simulink model "Hexapod_dev"  (R2026a)
settings: Solver=daessc  StopTime=ref.t(end)  FixedStep=2e-5
InitFcn:
  | startup
model workspace: external: MATLAB File Hexapod_DataFile.m (data not in the file)
undefined symbols (not defined in the file): ref, robot, smiData, X, Y, Z
libraries: sm_lib x805, nesl_utility x43
(part 14 of 15)

== system Hexapod_dev/Spherical Joints/HeimJoint_No_Ball_1_RIGID4/x6960T432_Super_Swivel_Ball_Joint_Rod_End_No_Ball_1_RIGID ==
  ReferenceFrame : sm_lib/Frames and Transforms/Reference Frame
  Solid : sm_lib/Body Elements/File Solid  ExtGeomFileName=6960T432_Super-Swivel Ball Joint Rod End No Ball_6960T432_sldprt.STEP  UnitType=FromFile  ExtGeomFileUnits=m  StepReaderType=HEX  ExportConvexHullGeometry=off  InertiaType=Custom  BasedOnType=DensityFromFile  Density=1000  DensityUnits=kg/m^3  Mass=smiData.Solid(21).mass  MassUnits=kg  CenterOfMass=smiData.Solid(21).CoM  CenterOfMassUnits=in  MomentsOfInertia=smiData.Solid(21).MoI  MomentsOfInertiaUnits=kg*in^2  ProductsOfInertia=smiData.Solid(21).PoI  ProductsOfInertiaUnits=kg*in^2  GraphicType=FromGeometry  MarkerShape=Sphere  MarkerSize=10  GraphicVisPropType=SimpleVisualProperties  GraphicDiffuseColor=smiData.Solid(21).color  GraphicOpacity=smiData.Solid(21).opacity  GraphicSpecularColor=[0.5 0.5 0.5 1.0]  GraphicAmbientColor=[0.15 0.15 0.15 1.0]  GraphicEmissiveColor=[0.0 0.0 0.0 1.0]  GraphicShininess=75  DoExposeReferenceFrame=on  SerializedFrames=|
      | <Frames>
      | 
      |   <Frame>
      |     <Id>Frame1</Id>
      |     <Value>
      |       <Name>T</Name>
      |       <Origin>
      |         <Source>GeometricFeature</Source>
      |         <FeatureName>spherical surface 2</FeatureName>
      |       </Origin>
      |       <PrimaryAxis>
      |         <DefinedDirection>+Z</DefinedDirection>
      |         <Source>ReferenceFrame</Source>
      |         <SourceDirection>+Z</SourceDirection>
      |         <FeatureName></FeatureName>
      |       </PrimaryAxis>
      |       <SecondaryAxis>
      |         <DefinedDirection>+X</DefinedDirection>
      |         <Source>GeometricFeature</Source>
      |         <SourceDirection>+X</SourceDirection>
      |         <FeatureName>segment 75</FeatureName>
      |       </SecondaryAxis>
      |     </Value>
      |   </Frame>
      | 
      | </Frames>
  F : PMIOPort  Side=Left
  T : PMIOPort  Port=2  Side=Left
  connections:
  ReferenceFrame/RConn1 -- Solid/RConn1 -- F/RConn1
  T/RConn1 -- Solid/LConn1

== system Hexapod_dev/Spherical Joints/HeimJoint_No_Ball_1_RIGID4/x8422N111_18_8_Stainless_Steel_Turnbuckle_Style_Connecting_Rod_1_RIGID ==
  ReferenceFrame : sm_lib/Frames and Transforms/Reference Frame
  Solid : sm_lib/Body Elements/File Solid  ExtGeomFileName=8422N111_18-8 Stainless Steel Turnbuckle-Style Connecting Rod_8422N111_sldprt.STEP  UnitType=FromFile  ExtGeomFileUnits=m  StepReaderType=HEX  ExportConvexHullGeometry=off  InertiaType=Custom  BasedOnType=DensityFromFile  Density=1000  DensityUnits=kg/m^3  Mass=smiData.Solid(19).mass  MassUnits=kg  CenterOfMass=smiData.Solid(19).CoM  CenterOfMassUnits=in  MomentsOfInertia=smiData.Solid(19).MoI  MomentsOfInertiaUnits=kg*in^2  ProductsOfInertia=smiData.Solid(19).PoI  ProductsOfInertiaUnits=kg*in^2  GraphicType=FromGeometry  MarkerShape=Sphere  MarkerSize=10  GraphicVisPropType=SimpleVisualProperties  GraphicDiffuseColor=smiData.Solid(19).color  GraphicOpacity=smiData.Solid(19).opacity  GraphicSpecularColor=[0.5 0.5 0.5 1.0]  GraphicAmbientColor=[0.15 0.15 0.15 1.0]  GraphicEmissiveColor=[0.0 0.0 0.0 1.0]  GraphicShininess=75  DoExposeReferenceFrame=on  SerializedFrames=<Frames/>
  F : PMIOPort  Side=Left
  connections:
  Solid/RConn1 -- ReferenceFrame/RConn1 -- F/RConn1

== system Hexapod_dev/Spherical Joints/HeimJoint_No_Ball_1_RIGID5/x6960T431_Super_Swivel_Ball_Joint_Rod_End_No_Ball_1_RIGID ==
  ReferenceFrame : sm_lib/Frames and Transforms/Reference Frame
  Solid : sm_lib/Body Elements/File Solid  ExtGeomFileName=6960T431_Super-Swivel Ball Joint Rod End No Ball_6960T431_sldprt.STEP  UnitType=FromFile  ExtGeomFileUnits=m  StepReaderType=HEX  ExportConvexHullGeometry=off  InertiaType=Custom  BasedOnType=DensityFromFile  Density=1000  DensityUnits=kg/m^3  Mass=smiData.Solid(20).mass  MassUnits=kg  CenterOfMass=smiData.Solid(20).CoM  CenterOfMassUnits=in  MomentsOfInertia=smiData.Solid(20).MoI  MomentsOfInertiaUnits=kg*in^2  ProductsOfInertia=smiData.Solid(20).PoI  ProductsOfInertiaUnits=kg*in^2  GraphicType=FromGeometry  MarkerShape=Sphere  MarkerSize=10  GraphicVisPropType=SimpleVisualProperties  GraphicDiffuseColor=smiData.Solid(20).color  GraphicOpacity=smiData.Solid(20).opacity  GraphicSpecularColor=[0.5 0.5 0.5 1.0]  GraphicAmbientColor=[0.15 0.15 0.15 1.0]  GraphicEmissiveColor=[0.0 0.0 0.0 1.0]  GraphicShininess=75  DoExposeReferenceFrame=on  SerializedFrames=|
      | <Frames>
      | 
      |   <Frame>
      |     <Id>Frame1</Id>
      |     <Value>
      |       <Name>B</Name>
      |       <Origin>
      |         <Source>GeometricFeature</Source>
      |         <FeatureName>circular curve 99</FeatureName>
      |       </Origin>
      |       <PrimaryAxis>
      |         <DefinedDirection>+Z</DefinedDirection>
      |         <Source>ReferenceFrame</Source>
      |         <SourceDirection>+Z</SourceDirection>
      |         <FeatureName></FeatureName>
      |       </PrimaryAxis>
      |       <SecondaryAxis>
      |         <DefinedDirection>-X</DefinedDirection>
      |         <Source>GeometricFeature</Source>
      |         <SourceDirection>+X</SourceDirection>
      |         <FeatureName>segment 73</FeatureName>
      |       </SecondaryAxis>
      |     </Value>
      |   </Frame>
      | 
      | </Frames>
  F : PMIOPort  Side=Left
  BO : PMIOPort  Port=2  Side=Left
  connections:
  ReferenceFrame/RConn1 -- Solid/RConn1 -- F/RConn1
  BO/RConn1 -- Solid/LConn1

== system Hexapod_dev/Spherical Joints/HeimJoint_No_Ball_1_RIGID5/x6960T432_Super_Swivel_Ball_Joint_Rod_End_No_Ball_1_RIGID ==
  ReferenceFrame : sm_lib/Frames and Transforms/Reference Frame
  Solid : sm_lib/Body Elements/File Solid  ExtGeomFileName=6960T432_Super-Swivel Ball Joint Rod End No Ball_6960T432_sldprt.STEP  UnitType=FromFile  ExtGeomFileUnits=m  StepReaderType=HEX  ExportConvexHullGeometry=off  InertiaType=Custom  BasedOnType=DensityFromFile  Density=1000  DensityUnits=kg/m^3  Mass=smiData.Solid(21).mass  MassUnits=kg  CenterOfMass=smiData.Solid(21).CoM  CenterOfMassUnits=in  MomentsOfInertia=smiData.Solid(21).MoI  MomentsOfInertiaUnits=kg*in^2  ProductsOfInertia=smiData.Solid(21).PoI  ProductsOfInertiaUnits=kg*in^2  GraphicType=FromGeometry  MarkerShape=Sphere  MarkerSize=10  GraphicVisPropType=SimpleVisualProperties  GraphicDiffuseColor=smiData.Solid(21).color  GraphicOpacity=smiData.Solid(21).opacity  GraphicSpecularColor=[0.5 0.5 0.5 1.0]  GraphicAmbientColor=[0.15 0.15 0.15 1.0]  GraphicEmissiveColor=[0.0 0.0 0.0 1.0]  GraphicShininess=75  DoExposeReferenceFrame=on  SerializedFrames=|
      | <Frames>
      | 
      |   <Frame>
      |     <Id>Frame1</Id>
      |     <Value>
      |       <Name>T</Name>
      |       <Origin>
      |         <Source>GeometricFeature</Source>
      |         <FeatureName>spherical surface 2</FeatureName>
      |       </Origin>
      |       <PrimaryAxis>
      |         <DefinedDirection>+Z</DefinedDirection>
      |         <Source>ReferenceFrame</Source>
      |         <SourceDirection>+Z</SourceDirection>
      |         <FeatureName></FeatureName>
      |       </PrimaryAxis>
      |       <SecondaryAxis>
      |         <DefinedDirection>+X</DefinedDirection>
      |         <Source>GeometricFeature</Source>
      |         <SourceDirection>+X</SourceDirection>
      |         <FeatureName>segment 75</FeatureName>
      |       </SecondaryAxis>
      |     </Value>
      |   </Frame>
      | 
      | </Frames>
  F : PMIOPort  Side=Left
  T : PMIOPort  Port=2  Side=Left
  connections:
  ReferenceFrame/RConn1 -- Solid/RConn1 -- F/RConn1
  T/RConn1 -- Solid/LConn1

== system Hexapod_dev/Spherical Joints/HeimJoint_No_Ball_1_RIGID5/x8422N111_18_8_Stainless_Steel_Turnbuckle_Style_Connecting_Rod_1_RIGID ==
  ReferenceFrame : sm_lib/Frames and Transforms/Reference Frame
  Solid : sm_lib/Body Elements/File Solid  ExtGeomFileName=8422N111_18-8 Stainless Steel Turnbuckle-Style Connecting Rod_8422N111_sldprt.STEP  UnitType=FromFile  ExtGeomFileUnits=m  StepReaderType=HEX  ExportConvexHullGeometry=off  InertiaType=Custom  BasedOnType=DensityFromFile  Density=1000  DensityUnits=kg/m^3  Mass=smiData.Solid(19).mass  MassUnits=kg  CenterOfMass=smiData.Solid(19).CoM  CenterOfMassUnits=in  MomentsOfInertia=smiData.Solid(19).MoI  MomentsOfInertiaUnits=kg*in^2  ProductsOfInertia=smiData.Solid(19).PoI  ProductsOfInertiaUnits=kg*in^2  GraphicType=FromGeometry  MarkerShape=Sphere  MarkerSize=10  GraphicVisPropType=SimpleVisualProperties  GraphicDiffuseColor=smiData.Solid(19).color  GraphicOpacity=smiData.Solid(19).opacity  GraphicSpecularColor=[0.5 0.5 0.5 1.0]  GraphicAmbientColor=[0.15 0.15 0.15 1.0]  GraphicEmissiveColor=[0.0 0.0 0.0 1.0]  GraphicShininess=75  DoExposeReferenceFrame=on  SerializedFrames=<Frames/>
  F : PMIOPort  Side=Left
  connections:
  Solid/RConn1 -- ReferenceFrame/RConn1 -- F/RConn1

== system Hexapod_dev/Spherical Joints/HeimJoint_No_Ball_1_RIGID6/x6960T431_Super_Swivel_Ball_Joint_Rod_End_No_Ball_1_RIGID ==
  ReferenceFrame : sm_lib/Frames and Transforms/Reference Frame
  Solid : sm_lib/Body Elements/File Solid  ExtGeomFileName=6960T431_Super-Swivel Ball Joint Rod End No Ball_6960T431_sldprt.STEP  UnitType=FromFile  ExtGeomFileUnits=m  StepReaderType=HEX  ExportConvexHullGeometry=off  InertiaType=Custom  BasedOnType=DensityFromFile  Density=1000  DensityUnits=kg/m^3  Mass=smiData.Solid(20).mass  MassUnits=kg  CenterOfMass=smiData.Solid(20).CoM  CenterOfMassUnits=in  MomentsOfInertia=smiData.Solid(20).MoI  MomentsOfInertiaUnits=kg*in^2  ProductsOfInertia=smiData.Solid(20).PoI  ProductsOfInertiaUnits=kg*in^2  GraphicType=FromGeometry  MarkerShape=Sphere  MarkerSize=10  GraphicVisPropType=SimpleVisualProperties  GraphicDiffuseColor=smiData.Solid(20).color  GraphicOpacity=smiData.Solid(20).opacity  GraphicSpecularColor=[0.5 0.5 0.5 1.0]  GraphicAmbientColor=[0.15 0.15 0.15 1.0]  GraphicEmissiveColor=[0.0 0.0 0.0 1.0]  GraphicShininess=75  DoExposeReferenceFrame=on  SerializedFrames=|
      | <Frames>
      | 
      |   <Frame>
      |     <Id>Frame1</Id>
      |     <Value>
      |       <Name>B</Name>
      |       <Origin>
      |         <Source>GeometricFeature</Source>
      |         <FeatureName>circular curve 99</FeatureName>
      |       </Origin>
      |       <PrimaryAxis>
      |         <DefinedDirection>+Z</DefinedDirection>
      |         <Source>ReferenceFrame</Source>
      |         <SourceDirection>+Z</SourceDirection>
      |         <FeatureName></FeatureName>
      |       </PrimaryAxis>
      |       <SecondaryAxis>
      |         <DefinedDirection>-X</DefinedDirection>
      |         <Source>GeometricFeature</Source>
      |         <SourceDirection>+X</SourceDirection>
      |         <FeatureName>segment 73</FeatureName>
      |       </SecondaryAxis>
      |     </Value>
      |   </Frame>
      | 
      | </Frames>
  F : PMIOPort  Side=Left
  B : PMIOPort  Port=2  Side=Right
  connections:
  ReferenceFrame/RConn1 -- Solid/RConn1 -- F/RConn1
  B/RConn1 -- Solid/LConn1

== system Hexapod_dev/Spherical Joints/HeimJoint_No_Ball_1_RIGID6/x6960T432_Super_Swivel_Ball_Joint_Rod_End_No_Ball_1_RIGID ==
  ReferenceFrame : sm_lib/Frames and Transforms/Reference Frame
  Solid : sm_lib/Body Elements/File Solid  ExtGeomFileName=6960T432_Super-Swivel Ball Joint Rod End No Ball_6960T432_sldprt.STEP  UnitType=FromFile  ExtGeomFileUnits=m  StepReaderType=HEX  ExportConvexHullGeometry=off  InertiaType=Custom  BasedOnType=DensityFromFile  Density=1000  DensityUnits=kg/m^3  Mass=smiData.Solid(21).mass  MassUnits=kg  CenterOfMass=smiData.Solid(21).CoM  CenterOfMassUnits=in  MomentsOfInertia=smiData.Solid(21).MoI  MomentsOfInertiaUnits=kg*in^2  ProductsOfInertia=smiData.Solid(21).PoI  ProductsOfInertiaUnits=kg*in^2  GraphicType=FromGeometry  MarkerShape=Sphere  MarkerSize=10  GraphicVisPropType=SimpleVisualProperties  GraphicDiffuseColor=smiData.Solid(21).color  GraphicOpacity=smiData.Solid(21).opacity  GraphicSpecularColor=[0.5 0.5 0.5 1.0]  GraphicAmbientColor=[0.15 0.15 0.15 1.0]  GraphicEmissiveColor=[0.0 0.0 0.0 1.0]  GraphicShininess=75  DoExposeReferenceFrame=on  SerializedFrames=|
      | <Frames>
      | 
      |   <Frame>
      |     <Id>Frame1</Id>
      |     <Value>
      |       <Name>T</Name>
      |       <Origin>
      |         <Source>GeometricFeature</Source>
      |         <FeatureName>spherical surface 2</FeatureName>
      |       </Origin>
      |       <PrimaryAxis>
      |         <DefinedDirection>+Z</DefinedDirection>
      |         <Source>ReferenceFrame</Source>
      |         <SourceDirection>+Z</SourceDirection>
      |         <FeatureName></FeatureName>
      |       </PrimaryAxis>
      |       <SecondaryAxis>
      |         <DefinedDirection>+X</DefinedDirection>
      |         <Source>GeometricFeature</Source>
      |         <SourceDirection>+X</SourceDirection>
      |         <FeatureName>segment 75</FeatureName>
      |       </SecondaryAxis>
      |     </Value>
      |   </Frame>
      | 
      | </Frames>
  F : PMIOPort  Side=Left
  T : PMIOPort  Port=2  Side=Right
  connections:
  ReferenceFrame/RConn1 -- Solid/RConn1 -- F/RConn1
  T/RConn1 -- Solid/LConn1

== system Hexapod_dev/Spherical Joints/HeimJoint_No_Ball_1_RIGID6/x8422N111_18_8_Stainless_Steel_Turnbuckle_Style_Connecting_Rod_1_RIGID ==
  ReferenceFrame : sm_lib/Frames and Transforms/Reference Frame
  Solid : sm_lib/Body Elements/File Solid  ExtGeomFileName=8422N111_18-8 Stainless Steel Turnbuckle-Style Connecting Rod_8422N111_sldprt.STEP  UnitType=FromFile  ExtGeomFileUnits=m  StepReaderType=HEX  ExportConvexHullGeometry=off  InertiaType=Custom  BasedOnType=DensityFromFile  Density=1000  DensityUnits=kg/m^3  Mass=smiData.Solid(19).mass  MassUnits=kg  CenterOfMass=smiData.Solid(19).CoM  CenterOfMassUnits=in  MomentsOfInertia=smiData.Solid(19).MoI  MomentsOfInertiaUnits=kg*in^2  ProductsOfInertia=smiData.Solid(19).PoI  ProductsOfInertiaUnits=kg*in^2  GraphicType=FromGeometry  MarkerShape=Sphere  MarkerSize=10  GraphicVisPropType=SimpleVisualProperties  GraphicDiffuseColor=smiData.Solid(19).color  GraphicOpacity=smiData.Solid(19).opacity  GraphicSpecularColor=[0.5 0.5 0.5 1.0]  GraphicAmbientColor=[0.15 0.15 0.15 1.0]  GraphicEmissiveColor=[0.0 0.0 0.0 1.0]  GraphicShininess=75  DoExposeReferenceFrame=on  SerializedFrames=<Frames/>
  F : PMIOPort  Side=Left
  connections:
  Solid/RConn1 -- ReferenceFrame/RConn1 -- F/RConn1

== system Hexapod_dev/Spherical Joints/MotorRotor_a_1_RIGID/MotorRotor_1_RIGID ==
  Inertia : sm_lib/Body Elements/Inertia  InertiaType=Custom  Mass=0  MassUnits=kg  CenterOfMass=[0 0 0]  CenterOfMassUnits=m  MomentsOfInertia="[0 0  robot.motor.reflectedInertia]"  MomentsOfInertiaUnits=kg*m^2  ProductsOfInertia=[0 0 0]  ProductsOfInertiaUnits=kg*m^2  GraphicType=None  MarkerShape=Inertia  MarkerSize=20  GraphicVisPropType=SimpleVisualProperties  GraphicDiffuseColor=[0.5 0.5 0.5]  GraphicOpacity=1  GraphicSpecularColor=[0.5 0.5 0.5 1.0]  GraphicAmbientColor=[0.15 0.15 0.15 1.0]  GraphicEmissiveColor=[0.0 0.0 0.0 1.0]  GraphicShininess=75
  ReferenceFrame : sm_lib/Frames and Transforms/Reference Frame
  Solid : sm_lib/Body Elements/File Solid  ExtGeomFileName=MotorRotor_Default_sldprt.STEP  UnitType=FromFile  ExtGeomFileUnits=m  StepReaderType=HEX  ExportConvexHullGeometry=off  InertiaType=Custom  BasedOnType=DensityFromFile  Density=1000  DensityUnits=kg/m^3  Mass=smiData.Solid(16).mass  MassUnits=kg  CenterOfMass=smiData.Solid(16).CoM  CenterOfMassUnits=mm  MomentsOfInertia=smiData.Solid(16).MoI  MomentsOfInertiaUnits=kg*mm^2  ProductsOfInertia=smiData.Solid(16).PoI  ProductsOfInertiaUnits=kg*mm^2  GraphicType=FromGeometry  MarkerShape=Sphere  MarkerSize=10  GraphicVisPropType=SimpleVisualProperties  GraphicDiffuseColor=smiData.Solid(16).color  GraphicOpacity=smiData.Solid(16).opacity  GraphicSpecularColor=[0.5 0.5 0.5 1.0]  GraphicAmbientColor=[0.15 0.15 0.15 1.0]  GraphicEmissiveColor=[0.0 0.0 0.0 1.0]  GraphicShininess=75  DoExposeReferenceFrame=on  SerializedFrames=<Frames/>
  F : PMIOPort  Side=Left
  connections:
  ReferenceFrame/RConn1 -- F/RConn1 -- Inertia/RConn1 -- Solid/RConn1

== system Hexapod_dev/Spherical Joints/MotorRotor_a_1_RIGID/ServoArm_1_RIGID ==
  ReferenceFrame : sm_lib/Frames and Transforms/Reference Frame
  Solid : sm_lib/Body Elements/File Solid  ExtGeomFileName=ServoArm_Default_sldprt.STEP  UnitType=FromFile  ExtGeomFileUnits=m  StepReaderType=HEX  ExportConvexHullGeometry=off  InertiaType=Custom  BasedOnType=DensityFromFile  Density=1000  DensityUnits=kg/m^3  Mass=smiData.Solid(18).mass  MassUnits=kg  CenterOfMass=smiData.Solid(18).CoM  CenterOfMassUnits=in  MomentsOfInertia=smiData.Solid(18).MoI  MomentsOfInertiaUnits=kg*in^2  ProductsOfInertia=smiData.Solid(18).PoI  ProductsOfInertiaUnits=kg*in^2  GraphicType=FromGeometry  MarkerShape=Sphere  MarkerSize=10  GraphicVisPropType=SimpleVisualProperties  GraphicDiffuseColor=smiData.Solid(18).color  GraphicOpacity=smiData.Solid(18).opacity  GraphicSpecularColor=[0.5 0.5 0.5 1.0]  GraphicAmbientColor=[0.15 0.15 0.15 1.0]  GraphicEmissiveColor=[0.0 0.0 0.0 1.0]  GraphicShininess=75  DoExposeReferenceFrame=on  SerializedFrames=<Frames/>
  F : PMIOPort  Side=Left
  connections:
  Solid/RConn1 -- ReferenceFrame/RConn1 -- F/RConn1

== system Hexapod_dev/Spherical Joints/MotorRotor_a_1_RIGID/ball_1_RIGID ==
  ReferenceFrame : sm_lib/Frames and Transforms/Reference Frame
  Solid : sm_lib/Body Elements/File Solid  ExtGeomFileName=ball_6960T431_sldprt.STEP  UnitType=FromFile  ExtGeomFileUnits=m  StepReaderType=HEX  ExportConvexHullGeometry=off  InertiaType=Custom  BasedOnType=DensityFromFile  Density=1000  DensityUnits=kg/m^3  Mass=smiData.Solid(12).mass  MassUnits=kg  CenterOfMass=smiData.Solid(12).CoM  CenterOfMassUnits=in  MomentsOfInertia=smiData.Solid(12).MoI  MomentsOfInertiaUnits=kg*in^2  ProductsOfInertia=smiData.Solid(12).PoI  ProductsOfInertiaUnits=kg*in^2  GraphicType=FromGeometry  MarkerShape=Sphere  MarkerSize=10  GraphicVisPropType=SimpleVisualProperties  GraphicDiffuseColor=smiData.Solid(12).color  GraphicOpacity=smiData.Solid(12).opacity  GraphicSpecularColor=[0.5 0.5 0.5 1.0]  GraphicAmbientColor=[0.15 0.15 0.15 1.0]  GraphicEmissiveColor=[0.0 0.0 0.0 1.0]  GraphicShininess=75  DoExposeReferenceFrame=on  SerializedFrames=<Frames/>
  F : PMIOPort  Side=Left
  connections:
  Solid/RConn1 -- ReferenceFrame/RConn1 -- F/RConn1

== system Hexapod_dev/Spherical Joints/MotorRotor_a_1_RIGID/x90790A185_Black_Oxide_Steel_High_Heavy_Profile_Cap_Nut_1_RIGID ==
  ReferenceFrame : sm_lib/Frames and Transforms/Reference Frame
  Solid : sm_lib/Body Elements/File Solid  ExtGeomFileName=90790A185_Black-Oxide Steel High-Heavy-Profile Cap Nut_90790A185_sldprt.STEP  UnitType=FromFile  ExtGeomFileUnits=m  StepReaderType=HEX  ExportConvexHullGeometry=off  InertiaType=Custom  BasedOnType=DensityFromFile  Density=1000  DensityUnits=kg/m^3  Mass=smiData.Solid(13).mass  MassUnits=kg  CenterOfMass=smiData.Solid(13).CoM  CenterOfMassUnits=in  MomentsOfInertia=smiData.Solid(13).MoI  MomentsOfInertiaUnits=kg*in^2  ProductsOfInertia=smiData.Solid(13).PoI  ProductsOfInertiaUnits=kg*in^2  GraphicType=FromGeometry  MarkerShape=Sphere  MarkerSize=10  GraphicVisPropType=SimpleVisualProperties  GraphicDiffuseColor=smiData.Solid(13).color  GraphicOpacity=smiData.Solid(13).opacity  GraphicSpecularColor=[0.5 0.5 0.5 1.0]  GraphicAmbientColor=[0.15 0.15 0.15 1.0]  GraphicEmissiveColor=[0.0 0.0 0.0 1.0]  GraphicShininess=75  DoExposeReferenceFrame=on  SerializedFrames=<Frames/>
  F : PMIOPort  Side=Left
  connections:
  Solid/RConn1 -- ReferenceFrame/RConn1 -- F/RConn1

== system Hexapod_dev/Spherical Joints/MotorRotor_a_1_RIGID/x91259A628_Alloy_Steel_Shoulder_Screw_1_RIGID ==
  ReferenceFrame : sm_lib/Frames and Transforms/Reference Frame
  Solid : sm_lib/Body Elements/File Solid  ExtGeomFileName=91259A628_Alloy Steel Shoulder Screw_91259A628_sldprt.STEP  UnitType=FromFile  ExtGeomFileUnits=m  StepReaderType=HEX  ExportConvexHullGeometry=off  InertiaType=Custom  BasedOnType=DensityFromFile  Density=1000  DensityUnits=kg/m^3  Mass=smiData.Solid(15).mass  MassUnits=kg  CenterOfMass=smiData.Solid(15).CoM  CenterOfMassUnits=in  MomentsOfInertia=smiData.Solid(15).MoI  MomentsOfInertiaUnits=kg*in^2  ProductsOfInertia=smiData.Solid(15).PoI  ProductsOfInertiaUnits=kg*in^2  GraphicType=FromGeometry  MarkerShape=Sphere  MarkerSize=10  GraphicVisPropType=SimpleVisualProperties  GraphicDiffuseColor=smiData.Solid(15).color  GraphicOpacity=smiData.Solid(15).opacity  GraphicSpecularColor=[0.5 0.5 0.5 1.0]  GraphicAmbientColor=[0.15 0.15 0.15 1.0]  GraphicEmissiveColor=[0.0 0.0 0.0 1.0]  GraphicShininess=75  DoExposeReferenceFrame=on  SerializedFrames=<Frames/>
  F : PMIOPort  Side=Left
  connections:
  Solid/RConn1 -- ReferenceFrame/RConn1 -- F/RConn1

== system Hexapod_dev/Spherical Joints/MotorRotor_a_1_RIGID/x91273A784_Same_Size_Thread_18_8_Stainless_Steel_Shoulder_Screw_1_RIGID ==
  ReferenceFrame : sm_lib/Frames and Transforms/Reference Frame
  Solid : sm_lib/Body Elements/File Solid  ExtGeomFileName=91273A784_Same-Size Thread 18-8 Stainless Steel Shoulder Screw_91273A784_sldprt.STEP  UnitType=FromFile  ExtGeomFileUnits=m  StepReaderType=HEX  ExportConvexHullGeometry=off  InertiaType=Custom  BasedOnType=DensityFromFile  Density=1000  DensityUnits=kg/m^3  Mass=smiData.Solid(10).mass  MassUnits=kg  CenterOfMass=smiData.Solid(10).CoM  CenterOfMassUnits=mm  MomentsOfInertia=smiData.Solid(10).MoI  MomentsOfInertiaUnits=kg*mm^2  ProductsOfInertia=smiData.Solid(10).PoI  ProductsOfInertiaUnits=kg*mm^2  GraphicType=FromGeometry  MarkerShape=Sphere  MarkerSize=10  GraphicVisPropType=SimpleVisualProperties  GraphicDiffuseColor=smiData.Solid(10).color  GraphicOpacity=smiData.Solid(10).opacity  GraphicSpecularColor=[0.5 0.5 0.5 1.0]  GraphicAmbientColor=[0.15 0.15 0.15 1.0]  GraphicEmissiveColor=[0.0 0.0 0.0 1.0]  GraphicShininess=75  DoExposeReferenceFrame=on  SerializedFrames=<Frames/>
  F : PMIOPort  Side=Left
  connections:
  Solid/RConn1 -- ReferenceFrame/RConn1 -- F/RConn1

== system Hexapod_dev/Spherical Joints/MotorRotor_a_1_RIGID/x91273A784_Same_Size_Thread_18_8_Stainless_Steel_Shoulder_Screw_2_RIGID ==
  ReferenceFrame : sm_lib/Frames and Transforms/Reference Frame
  Solid : sm_lib/Body Elements/File Solid  ExtGeomFileName=91273A784_Same-Size Thread 18-8 Stainless Steel Shoulder Screw_91273A784_sldprt.STEP  UnitType=FromFile  ExtGeomFileUnits=m  StepReaderType=HEX  ExportConvexHullGeometry=off  InertiaType=Custom  BasedOnType=DensityFromFile  Density=1000  DensityUnits=kg/m^3  Mass=smiData.Solid(10).mass  MassUnits=kg  CenterOfMass=smiData.Solid(10).CoM  CenterOfMassUnits=mm  MomentsOfInertia=smiData.Solid(10).MoI  MomentsOfInertiaUnits=kg*mm^2  ProductsOfInertia=smiData.Solid(10).PoI  ProductsOfInertiaUnits=kg*mm^2  GraphicType=FromGeometry  MarkerShape=Sphere  MarkerSize=10  GraphicVisPropType=SimpleVisualProperties  GraphicDiffuseColor=smiData.Solid(10).color  GraphicOpacity=smiData.Solid(10).opacity  GraphicSpecularColor=[0.5 0.5 0.5 1.0]  GraphicAmbientColor=[0.15 0.15 0.15 1.0]  GraphicEmissiveColor=[0.0 0.0 0.0 1.0]  GraphicShininess=75  DoExposeReferenceFrame=on  SerializedFrames=<Frames/>
  F : PMIOPort  Side=Left
  connections:
  Solid/RConn1 -- ReferenceFrame/RConn1 -- F/RConn1

== system Hexapod_dev/Spherical Joints/MotorRotor_a_1_RIGID/x91273A784_Same_Size_Thread_18_8_Stainless_Steel_Shoulder_Screw_3_RIGID ==
  ReferenceFrame : sm_lib/Frames and Transforms/Reference Frame
  Solid : sm_lib/Body Elements/File Solid  ExtGeomFileName=91273A784_Same-Size Thread 18-8 Stainless Steel Shoulder Screw_91273A784_sldprt.STEP  UnitType=FromFile  ExtGeomFileUnits=m  StepReaderType=HEX  ExportConvexHullGeometry=off  InertiaType=Custom  BasedOnType=DensityFromFile  Density=1000  DensityUnits=kg/m^3  Mass=smiData.Solid(10).mass  MassUnits=kg  CenterOfMass=smiData.Solid(10).CoM  CenterOfMassUnits=mm  MomentsOfInertia=smiData.Solid(10).MoI  MomentsOfInertiaUnits=kg*mm^2  ProductsOfInertia=smiData.Solid(10).PoI  ProductsOfInertiaUnits=kg*mm^2  GraphicType=FromGeometry  MarkerShape=Sphere  MarkerSize=10  GraphicVisPropType=SimpleVisualProperties  GraphicDiffuseColor=smiData.Solid(10).color  GraphicOpacity=smiData.Solid(10).opacity  GraphicSpecularColor=[0.5 0.5 0.5 1.0]  GraphicAmbientColor=[0.15 0.15 0.15 1.0]  GraphicEmissiveColor=[0.0 0.0 0.0 1.0]  GraphicShininess=75  DoExposeReferenceFrame=on  SerializedFrames=<Frames/>
  F : PMIOPort  Side=Left
  connections:
  Solid/RConn1 -- ReferenceFrame/RConn1 -- F/RConn1

== system Hexapod_dev/Spherical Joints/MotorRotor_a_1_RIGID/x92510A494_Aluminum_Unthreaded_Spacer_1_RIGID ==
  ReferenceFrame : sm_lib/Frames and Transforms/Reference Frame
  Solid : sm_lib/Body Elements/File Solid  ExtGeomFileName=92510A494_Aluminum Unthreaded Spacer_92510A494_sldprt.STEP  UnitType=FromFile  ExtGeomFileUnits=m  StepReaderType=HEX  ExportConvexHullGeometry=off  InertiaType=Custom  BasedOnType=DensityFromFile  Density=1000  DensityUnits=kg/m^3  Mass=smiData.Solid(17).mass  MassUnits=kg  CenterOfMass=smiData.Solid(17).CoM  CenterOfMassUnits=in  MomentsOfInertia=smiData.Solid(17).MoI  MomentsOfInertiaUnits=kg*in^2  ProductsOfInertia=smiData.Solid(17).PoI  ProductsOfInertiaUnits=kg*in^2  GraphicType=FromGeometry  MarkerShape=Sphere  MarkerSize=10  GraphicVisPropType=SimpleVisualProperties  GraphicDiffuseColor=smiData.Solid(17).color  GraphicOpacity=smiData.Solid(17).opacity  GraphicSpecularColor=[0.5 0.5 0.5 1.0]  GraphicAmbientColor=[0.15 0.15 0.15 1.0]  GraphicEmissiveColor=[0.0 0.0 0.0 1.0]  GraphicShininess=75  DoExposeReferenceFrame=on  SerializedFrames=<Frames/>
  F : PMIOPort  Side=Left
  connections:
  Solid/RConn1 -- ReferenceFrame/RConn1 -- F/RConn1

== system Hexapod_dev/Spherical Joints/MotorRotor_a_1_RIGID/x93413A312_Black_Super_Corrosion_Resistant_Coated_Steel_Washer_1_RIGID ==
  ReferenceFrame : sm_lib/Frames and Transforms/Reference Frame
  Solid : sm_lib/Body Elements/File Solid  ExtGeomFileName=93413A312_Black Super-Corrosion-Resistant-Coated Steel Washer_93413A312_sldprt.STEP  UnitType=FromFile  ExtGeomFileUnits=m  StepReaderType=HEX  ExportConvexHullGeometry=off  InertiaType=Custom  BasedOnType=DensityFromFile  Density=1000  DensityUnits=kg/m^3  Mass=smiData.Solid(14).mass  MassUnits=kg  CenterOfMass=smiData.Solid(14).CoM  CenterOfMassUnits=in  MomentsOfInertia=smiData.Solid(14).MoI  MomentsOfInertiaUnits=kg*in^2  ProductsOfInertia=smiData.Solid(14).PoI  ProductsOfInertiaUnits=kg*in^2  GraphicType=FromGeometry  MarkerShape=Sphere  MarkerSize=10  GraphicVisPropType=SimpleVisualProperties  GraphicDiffuseColor=smiData.Solid(14).color  GraphicOpacity=smiData.Solid(14).opacity  GraphicSpecularColor=[0.5 0.5 0.5 1.0]  GraphicAmbientColor=[0.15 0.15 0.15 1.0]  GraphicEmissiveColor=[0.0 0.0 0.0 1.0]  GraphicShininess=75  DoExposeReferenceFrame=on  SerializedFrames=<Frames/>
  F : PMIOPort  Side=Left
  connections:
  Solid/RConn1 -- ReferenceFrame/RConn1 -- F/RConn1

== system Hexapod_dev/Spherical Joints/MotorRotor_a_2_RIGID/MotorRotor_1_RIGID ==
  Inertia : sm_lib/Body Elements/Inertia  InertiaType=Custom  Mass=0  MassUnits=kg  CenterOfMass=[0 0 0]  CenterOfMassUnits=m  MomentsOfInertia="[0 0  robot.motor.reflectedInertia]"  MomentsOfInertiaUnits=kg*m^2  ProductsOfInertia=[0 0 0]  ProductsOfInertiaUnits=kg*m^2  GraphicType=None  MarkerShape=Inertia  MarkerSize=20  GraphicVisPropType=SimpleVisualProperties  GraphicDiffuseColor=[0.5 0.5 0.5]  GraphicOpacity=1  GraphicSpecularColor=[0.5 0.5 0.5 1.0]  GraphicAmbientColor=[0.15 0.15 0.15 1.0]  GraphicEmissiveColor=[0.0 0.0 0.0 1.0]  GraphicShininess=75
  ReferenceFrame : sm_lib/Frames and Transforms/Reference Frame
  Solid : sm_lib/Body Elements/File Solid  ExtGeomFileName=MotorRotor_Default_sldprt.STEP  UnitType=FromFile  ExtGeomFileUnits=m  StepReaderType=HEX  ExportConvexHullGeometry=off  InertiaType=Custom  BasedOnType=DensityFromFile  Density=1000  DensityUnits=kg/m^3  Mass=smiData.Solid(16).mass  MassUnits=kg  CenterOfMass=smiData.Solid(16).CoM  CenterOfMassUnits=mm  MomentsOfInertia=smiData.Solid(16).MoI  MomentsOfInertiaUnits=kg*mm^2  ProductsOfInertia=smiData.Solid(16).PoI  ProductsOfInertiaUnits=kg*mm^2  GraphicType=FromGeometry  MarkerShape=Sphere  MarkerSize=10  GraphicVisPropType=SimpleVisualProperties  GraphicDiffuseColor=smiData.Solid(16).color  GraphicOpacity=smiData.Solid(16).opacity  GraphicSpecularColor=[0.5 0.5 0.5 1.0]  GraphicAmbientColor=[0.15 0.15 0.15 1.0]  GraphicEmissiveColor=[0.0 0.0 0.0 1.0]  GraphicShininess=75  DoExposeReferenceFrame=on  SerializedFrames=<Frames/>
  F : PMIOPort  Side=Left
  connections:
  ReferenceFrame/RConn1 -- F/RConn1 -- Inertia/RConn1 -- Solid/RConn1

== system Hexapod_dev/Spherical Joints/MotorRotor_a_2_RIGID/ServoArm_1_RIGID ==
  ReferenceFrame : sm_lib/Frames and Transforms/Reference Frame
  Solid : sm_lib/Body Elements/File Solid  ExtGeomFileName=ServoArm_Default_sldprt.STEP  UnitType=FromFile  ExtGeomFileUnits=m  StepReaderType=HEX  ExportConvexHullGeometry=off  InertiaType=Custom  BasedOnType=DensityFromFile  Density=1000  DensityUnits=kg/m^3  Mass=smiData.Solid(18).mass  MassUnits=kg  CenterOfMass=smiData.Solid(18).CoM  CenterOfMassUnits=in  MomentsOfInertia=smiData.Solid(18).MoI  MomentsOfInertiaUnits=kg*in^2  ProductsOfInertia=smiData.Solid(18).PoI  ProductsOfInertiaUnits=kg*in^2  GraphicType=FromGeometry  MarkerShape=Sphere  MarkerSize=10  GraphicVisPropType=SimpleVisualProperties  GraphicDiffuseColor=smiData.Solid(18).color  GraphicOpacity=smiData.Solid(18).opacity  GraphicSpecularColor=[0.5 0.5 0.5 1.0]  GraphicAmbientColor=[0.15 0.15 0.15 1.0]  GraphicEmissiveColor=[0.0 0.0 0.0 1.0]  GraphicShininess=75  DoExposeReferenceFrame=on  SerializedFrames=<Frames/>
  F : PMIOPort  Side=Left
  connections:
  Solid/RConn1 -- ReferenceFrame/RConn1 -- F/RConn1

== system Hexapod_dev/Spherical Joints/MotorRotor_a_2_RIGID/ball_1_RIGID ==
  ReferenceFrame : sm_lib/Frames and Transforms/Reference Frame
  Solid : sm_lib/Body Elements/File Solid  ExtGeomFileName=ball_6960T431_sldprt.STEP  UnitType=FromFile  ExtGeomFileUnits=m  StepReaderType=HEX  ExportConvexHullGeometry=off  InertiaType=Custom  BasedOnType=DensityFromFile  Density=1000  DensityUnits=kg/m^3  Mass=smiData.Solid(12).mass  MassUnits=kg  CenterOfMass=smiData.Solid(12).CoM  CenterOfMassUnits=in  MomentsOfInertia=smiData.Solid(12).MoI  MomentsOfInertiaUnits=kg*in^2  ProductsOfInertia=smiData.Solid(12).PoI  ProductsOfInertiaUnits=kg*in^2  GraphicType=FromGeometry  MarkerShape=Sphere  MarkerSize=10  GraphicVisPropType=SimpleVisualProperties  GraphicDiffuseColor=smiData.Solid(12).color  GraphicOpacity=smiData.Solid(12).opacity  GraphicSpecularColor=[0.5 0.5 0.5 1.0]  GraphicAmbientColor=[0.15 0.15 0.15 1.0]  GraphicEmissiveColor=[0.0 0.0 0.0 1.0]  GraphicShininess=75  DoExposeReferenceFrame=on  SerializedFrames=<Frames/>
  F : PMIOPort  Side=Left
  connections:
  Solid/RConn1 -- ReferenceFrame/RConn1 -- F/RConn1

== system Hexapod_dev/Spherical Joints/MotorRotor_a_2_RIGID/x90790A185_Black_Oxide_Steel_High_Heavy_Profile_Cap_Nut_1_RIGID ==
  ReferenceFrame : sm_lib/Frames and Transforms/Reference Frame
  Solid : sm_lib/Body Elements/File Solid  ExtGeomFileName=90790A185_Black-Oxide Steel High-Heavy-Profile Cap Nut_90790A185_sldprt.STEP  UnitType=FromFile  ExtGeomFileUnits=m  StepReaderType=HEX  ExportConvexHullGeometry=off  InertiaType=Custom  BasedOnType=DensityFromFile  Density=1000  DensityUnits=kg/m^3  Mass=smiData.Solid(13).mass  MassUnits=kg  CenterOfMass=smiData.Solid(13).CoM  CenterOfMassUnits=in  MomentsOfInertia=smiData.Solid(13).MoI  MomentsOfInertiaUnits=kg*in^2  ProductsOfInertia=smiData.Solid(13).PoI  ProductsOfInertiaUnits=kg*in^2  GraphicType=FromGeometry  MarkerShape=Sphere  MarkerSize=10  GraphicVisPropType=SimpleVisualProperties  GraphicDiffuseColor=smiData.Solid(13).color  GraphicOpacity=smiData.Solid(13).opacity  GraphicSpecularColor=[0.5 0.5 0.5 1.0]  GraphicAmbientColor=[0.15 0.15 0.15 1.0]  GraphicEmissiveColor=[0.0 0.0 0.0 1.0]  GraphicShininess=75  DoExposeReferenceFrame=on  SerializedFrames=<Frames/>
  F : PMIOPort  Side=Left
  connections:
  Solid/RConn1 -- ReferenceFrame/RConn1 -- F/RConn1

== system Hexapod_dev/Spherical Joints/MotorRotor_a_2_RIGID/x91259A628_Alloy_Steel_Shoulder_Screw_1_RIGID ==
  ReferenceFrame : sm_lib/Frames and Transforms/Reference Frame
  Solid : sm_lib/Body Elements/File Solid  ExtGeomFileName=91259A628_Alloy Steel Shoulder Screw_91259A628_sldprt.STEP  UnitType=FromFile  ExtGeomFileUnits=m  StepReaderType=HEX  ExportConvexHullGeometry=off  InertiaType=Custom  BasedOnType=DensityFromFile  Density=1000  DensityUnits=kg/m^3  Mass=smiData.Solid(15).mass  MassUnits=kg  CenterOfMass=smiData.Solid(15).CoM  CenterOfMassUnits=in  MomentsOfInertia=smiData.Solid(15).MoI  MomentsOfInertiaUnits=kg*in^2  ProductsOfInertia=smiData.Solid(15).PoI  ProductsOfInertiaUnits=kg*in^2  GraphicType=FromGeometry  MarkerShape=Sphere  MarkerSize=10  GraphicVisPropType=SimpleVisualProperties  GraphicDiffuseColor=smiData.Solid(15).color  GraphicOpacity=smiData.Solid(15).opacity  GraphicSpecularColor=[0.5 0.5 0.5 1.0]  GraphicAmbientColor=[0.15 0.15 0.15 1.0]  GraphicEmissiveColor=[0.0 0.0 0.0 1.0]  GraphicShininess=75  DoExposeReferenceFrame=on  SerializedFrames=<Frames/>
  F : PMIOPort  Side=Left
  connections:
  Solid/RConn1 -- ReferenceFrame/RConn1 -- F/RConn1

== system Hexapod_dev/Spherical Joints/MotorRotor_a_2_RIGID/x91273A784_Same_Size_Thread_18_8_Stainless_Steel_Shoulder_Screw_1_RIGID ==
  ReferenceFrame : sm_lib/Frames and Transforms/Reference Frame
  Solid : sm_lib/Body Elements/File Solid  ExtGeomFileName=91273A784_Same-Size Thread 18-8 Stainless Steel Shoulder Screw_91273A784_sldprt.STEP  UnitType=FromFile  ExtGeomFileUnits=m  StepReaderType=HEX  ExportConvexHullGeometry=off  InertiaType=Custom  BasedOnType=DensityFromFile  Density=1000  DensityUnits=kg/m^3  Mass=smiData.Solid(10).mass  MassUnits=kg  CenterOfMass=smiData.Solid(10).CoM  CenterOfMassUnits=mm  MomentsOfInertia=smiData.Solid(10).MoI  MomentsOfInertiaUnits=kg*mm^2  ProductsOfInertia=smiData.Solid(10).PoI  ProductsOfInertiaUnits=kg*mm^2  GraphicType=FromGeometry  MarkerShape=Sphere  MarkerSize=10  GraphicVisPropType=SimpleVisualProperties  GraphicDiffuseColor=smiData.Solid(10).color  GraphicOpacity=smiData.Solid(10).opacity  GraphicSpecularColor=[0.5 0.5 0.5 1.0]  GraphicAmbientColor=[0.15 0.15 0.15 1.0]  GraphicEmissiveColor=[0.0 0.0 0.0 1.0]  GraphicShininess=75  DoExposeReferenceFrame=on  SerializedFrames=<Frames/>
  F : PMIOPort  Side=Left
  connections:
  Solid/RConn1 -- ReferenceFrame/RConn1 -- F/RConn1

== system Hexapod_dev/Spherical Joints/MotorRotor_a_2_RIGID/x91273A784_Same_Size_Thread_18_8_Stainless_Steel_Shoulder_Screw_2_RIGID ==
  ReferenceFrame : sm_lib/Frames and Transforms/Reference Frame
  Solid : sm_lib/Body Elements/File Solid  ExtGeomFileName=91273A784_Same-Size Thread 18-8 Stainless Steel Shoulder Screw_91273A784_sldprt.STEP  UnitType=FromFile  ExtGeomFileUnits=m  StepReaderType=HEX  ExportConvexHullGeometry=off  InertiaType=Custom  BasedOnType=DensityFromFile  Density=1000  DensityUnits=kg/m^3  Mass=smiData.Solid(10).mass  MassUnits=kg  CenterOfMass=smiData.Solid(10).CoM  CenterOfMassUnits=mm  MomentsOfInertia=smiData.Solid(10).MoI  MomentsOfInertiaUnits=kg*mm^2  ProductsOfInertia=smiData.Solid(10).PoI  ProductsOfInertiaUnits=kg*mm^2  GraphicType=FromGeometry  MarkerShape=Sphere  MarkerSize=10  GraphicVisPropType=SimpleVisualProperties  GraphicDiffuseColor=smiData.Solid(10).color  GraphicOpacity=smiData.Solid(10).opacity  GraphicSpecularColor=[0.5 0.5 0.5 1.0]  GraphicAmbientColor=[0.15 0.15 0.15 1.0]  GraphicEmissiveColor=[0.0 0.0 0.0 1.0]  GraphicShininess=75  DoExposeReferenceFrame=on  SerializedFrames=<Frames/>
  F : PMIOPort  Side=Left
  connections:
  Solid/RConn1 -- ReferenceFrame/RConn1 -- F/RConn1

== system Hexapod_dev/Spherical Joints/MotorRotor_a_2_RIGID/x91273A784_Same_Size_Thread_18_8_Stainless_Steel_Shoulder_Screw_3_RIGID ==
  ReferenceFrame : sm_lib/Frames and Transforms/Reference Frame
  Solid : sm_lib/Body Elements/File Solid  ExtGeomFileName=91273A784_Same-Size Thread 18-8 Stainless Steel Shoulder Screw_91273A784_sldprt.STEP  UnitType=FromFile  ExtGeomFileUnits=m  StepReaderType=HEX  ExportConvexHullGeometry=off  InertiaType=Custom  BasedOnType=DensityFromFile  Density=1000  DensityUnits=kg/m^3  Mass=smiData.Solid(10).mass  MassUnits=kg  CenterOfMass=smiData.Solid(10).CoM  CenterOfMassUnits=mm  MomentsOfInertia=smiData.Solid(10).MoI  MomentsOfInertiaUnits=kg*mm^2  ProductsOfInertia=smiData.Solid(10).PoI  ProductsOfInertiaUnits=kg*mm^2  GraphicType=FromGeometry  MarkerShape=Sphere  MarkerSize=10  GraphicVisPropType=SimpleVisualProperties  GraphicDiffuseColor=smiData.Solid(10).color  GraphicOpacity=smiData.Solid(10).opacity  GraphicSpecularColor=[0.5 0.5 0.5 1.0]  GraphicAmbientColor=[0.15 0.15 0.15 1.0]  GraphicEmissiveColor=[0.0 0.0 0.0 1.0]  GraphicShininess=75  DoExposeReferenceFrame=on  SerializedFrames=<Frames/>
  F : PMIOPort  Side=Left
  connections:
  Solid/RConn1 -- ReferenceFrame/RConn1 -- F/RConn1

== system Hexapod_dev/Spherical Joints/MotorRotor_a_2_RIGID/x92510A494_Aluminum_Unthreaded_Spacer_1_RIGID ==
  ReferenceFrame : sm_lib/Frames and Transforms/Reference Frame
  Solid : sm_lib/Body Elements/File Solid  ExtGeomFileName=92510A494_Aluminum Unthreaded Spacer_92510A494_sldprt.STEP  UnitType=FromFile  ExtGeomFileUnits=m  StepReaderType=HEX  ExportConvexHullGeometry=off  InertiaType=Custom  BasedOnType=DensityFromFile  Density=1000  DensityUnits=kg/m^3  Mass=smiData.Solid(17).mass  MassUnits=kg  CenterOfMass=smiData.Solid(17).CoM  CenterOfMassUnits=in  MomentsOfInertia=smiData.Solid(17).MoI  MomentsOfInertiaUnits=kg*in^2  ProductsOfInertia=smiData.Solid(17).PoI  ProductsOfInertiaUnits=kg*in^2  GraphicType=FromGeometry  MarkerShape=Sphere  MarkerSize=10  GraphicVisPropType=SimpleVisualProperties  GraphicDiffuseColor=smiData.Solid(17).color  GraphicOpacity=smiData.Solid(17).opacity  GraphicSpecularColor=[0.5 0.5 0.5 1.0]  GraphicAmbientColor=[0.15 0.15 0.15 1.0]  GraphicEmissiveColor=[0.0 0.0 0.0 1.0]  GraphicShininess=75  DoExposeReferenceFrame=on  SerializedFrames=<Frames/>
  F : PMIOPort  Side=Left
  connections:
  Solid/RConn1 -- ReferenceFrame/RConn1 -- F/RConn1

== system Hexapod_dev/Spherical Joints/MotorRotor_a_2_RIGID/x93413A312_Black_Super_Corrosion_Resistant_Coated_Steel_Washer_1_RIGID ==
  ReferenceFrame : sm_lib/Frames and Transforms/Reference Frame
  Solid : sm_lib/Body Elements/File Solid  ExtGeomFileName=93413A312_Black Super-Corrosion-Resistant-Coated Steel Washer_93413A312_sldprt.STEP  UnitType=FromFile  ExtGeomFileUnits=m  StepReaderType=HEX  ExportConvexHullGeometry=off  InertiaType=Custom  BasedOnType=DensityFromFile  Density=1000  DensityUnits=kg/m^3  Mass=smiData.Solid(14).mass  MassUnits=kg  CenterOfMass=smiData.Solid(14).CoM  CenterOfMassUnits=in  MomentsOfInertia=smiData.Solid(14).MoI  MomentsOfInertiaUnits=kg*in^2  ProductsOfInertia=smiData.Solid(14).PoI  ProductsOfInertiaUnits=kg*in^2  GraphicType=FromGeometry  MarkerShape=Sphere  MarkerSize=10  GraphicVisPropType=SimpleVisualProperties  GraphicDiffuseColor=smiData.Solid(14).color  GraphicOpacity=smiData.Solid(14).opacity  GraphicSpecularColor=[0.5 0.5 0.5 1.0]  GraphicAmbientColor=[0.15 0.15 0.15 1.0]  GraphicEmissiveColor=[0.0 0.0 0.0 1.0]  GraphicShininess=75  DoExposeReferenceFrame=on  SerializedFrames=<Frames/>
  F : PMIOPort  Side=Left
  connections:
  Solid/RConn1 -- ReferenceFrame/RConn1 -- F/RConn1

== system Hexapod_dev/Spherical Joints/MotorRotor_a_3_RIGID/MotorRotor_1_RIGID ==
  Inertia : sm_lib/Body Elements/Inertia  InertiaType=Custom  Mass=0  MassUnits=kg  CenterOfMass=[0 0 0]  CenterOfMassUnits=m  MomentsOfInertia="[0 0  robot.motor.reflectedInertia]"  MomentsOfInertiaUnits=kg*m^2  ProductsOfInertia=[0 0 0]  ProductsOfInertiaUnits=kg*m^2  GraphicType=None  MarkerShape=Inertia  MarkerSize=20  GraphicVisPropType=SimpleVisualProperties  GraphicDiffuseColor=[0.5 0.5 0.5]  GraphicOpacity=1  GraphicSpecularColor=[0.5 0.5 0.5 1.0]  GraphicAmbientColor=[0.15 0.15 0.15 1.0]  GraphicEmissiveColor=[0.0 0.0 0.0 1.0]  GraphicShininess=75
  ReferenceFrame : sm_lib/Frames and Transforms/Reference Frame
  Solid : sm_lib/Body Elements/File Solid  ExtGeomFileName=MotorRotor_Default_sldprt.STEP  UnitType=FromFile  ExtGeomFileUnits=m  StepReaderType=HEX  ExportConvexHullGeometry=off  InertiaType=Custom  BasedOnType=DensityFromFile  Density=1000  DensityUnits=kg/m^3  Mass=smiData.Solid(16).mass  MassUnits=kg  CenterOfMass=smiData.Solid(16).CoM  CenterOfMassUnits=mm  MomentsOfInertia=smiData.Solid(16).MoI  MomentsOfInertiaUnits=kg*mm^2  ProductsOfInertia=smiData.Solid(16).PoI  ProductsOfInertiaUnits=kg*mm^2  GraphicType=FromGeometry  MarkerShape=Sphere  MarkerSize=10  GraphicVisPropType=SimpleVisualProperties  GraphicDiffuseColor=smiData.Solid(16).color  GraphicOpacity=smiData.Solid(16).opacity  GraphicSpecularColor=[0.5 0.5 0.5 1.0]  GraphicAmbientColor=[0.15 0.15 0.15 1.0]  GraphicEmissiveColor=[0.0 0.0 0.0 1.0]  GraphicShininess=75  DoExposeReferenceFrame=on  SerializedFrames=<Frames/>
  F : PMIOPort  Side=Left
  connections:
  ReferenceFrame/RConn1 -- F/RConn1 -- Inertia/RConn1 -- Solid/RConn1

== system Hexapod_dev/Spherical Joints/MotorRotor_a_3_RIGID/ServoArm_1_RIGID ==
  ReferenceFrame : sm_lib/Frames and Transforms/Reference Frame
  Solid : sm_lib/Body Elements/File Solid  ExtGeomFileName=ServoArm_Default_sldprt.STEP  UnitType=FromFile  ExtGeomFileUnits=m  StepReaderType=HEX  ExportConvexHullGeometry=off  InertiaType=Custom  BasedOnType=DensityFromFile  Density=1000  DensityUnits=kg/m^3  Mass=smiData.Solid(18).mass  MassUnits=kg  CenterOfMass=smiData.Solid(18).CoM  CenterOfMassUnits=in  MomentsOfInertia=smiData.Solid(18).MoI  MomentsOfInertiaUnits=kg*in^2  ProductsOfInertia=smiData.Solid(18).PoI  ProductsOfInertiaUnits=kg*in^2  GraphicType=FromGeometry  MarkerShape=Sphere  MarkerSize=10  GraphicVisPropType=SimpleVisualProperties  GraphicDiffuseColor=smiData.Solid(18).color  GraphicOpacity=smiData.Solid(18).opacity  GraphicSpecularColor=[0.5 0.5 0.5 1.0]  GraphicAmbientColor=[0.15 0.15 0.15 1.0]  GraphicEmissiveColor=[0.0 0.0 0.0 1.0]  GraphicShininess=75  DoExposeReferenceFrame=on  SerializedFrames=<Frames/>
  F : PMIOPort  Side=Left
  connections:
  Solid/RConn1 -- ReferenceFrame/RConn1 -- F/RConn1

== system Hexapod_dev/Spherical Joints/MotorRotor_a_3_RIGID/ball_1_RIGID ==
  ReferenceFrame : sm_lib/Frames and Transforms/Reference Frame
  Solid : sm_lib/Body Elements/File Solid  ExtGeomFileName=ball_6960T431_sldprt.STEP  UnitType=FromFile  ExtGeomFileUnits=m  StepReaderType=HEX  ExportConvexHullGeometry=off  InertiaType=Custom  BasedOnType=DensityFromFile  Density=1000  DensityUnits=kg/m^3  Mass=smiData.Solid(12).mass  MassUnits=kg  CenterOfMass=smiData.Solid(12).CoM  CenterOfMassUnits=in  MomentsOfInertia=smiData.Solid(12).MoI  MomentsOfInertiaUnits=kg*in^2  ProductsOfInertia=smiData.Solid(12).PoI  ProductsOfInertiaUnits=kg*in^2  GraphicType=FromGeometry  MarkerShape=Sphere  MarkerSize=10  GraphicVisPropType=SimpleVisualProperties  GraphicDiffuseColor=smiData.Solid(12).color  GraphicOpacity=smiData.Solid(12).opacity  GraphicSpecularColor=[0.5 0.5 0.5 1.0]  GraphicAmbientColor=[0.15 0.15 0.15 1.0]  GraphicEmissiveColor=[0.0 0.0 0.0 1.0]  GraphicShininess=75  DoExposeReferenceFrame=on  SerializedFrames=<Frames/>
  F : PMIOPort  Side=Left
  connections:
  Solid/RConn1 -- ReferenceFrame/RConn1 -- F/RConn1

== system Hexapod_dev/Spherical Joints/MotorRotor_a_3_RIGID/x90790A185_Black_Oxide_Steel_High_Heavy_Profile_Cap_Nut_1_RIGID ==
  ReferenceFrame : sm_lib/Frames and Transforms/Reference Frame
  Solid : sm_lib/Body Elements/File Solid  ExtGeomFileName=90790A185_Black-Oxide Steel High-Heavy-Profile Cap Nut_90790A185_sldprt.STEP  UnitType=FromFile  ExtGeomFileUnits=m  StepReaderType=HEX  ExportConvexHullGeometry=off  InertiaType=Custom  BasedOnType=DensityFromFile  Density=1000  DensityUnits=kg/m^3  Mass=smiData.Solid(13).mass  MassUnits=kg  CenterOfMass=smiData.Solid(13).CoM  CenterOfMassUnits=in  MomentsOfInertia=smiData.Solid(13).MoI  MomentsOfInertiaUnits=kg*in^2  ProductsOfInertia=smiData.Solid(13).PoI  ProductsOfInertiaUnits=kg*in^2  GraphicType=FromGeometry  MarkerShape=Sphere  MarkerSize=10  GraphicVisPropType=SimpleVisualProperties  GraphicDiffuseColor=smiData.Solid(13).color  GraphicOpacity=smiData.Solid(13).opacity  GraphicSpecularColor=[0.5 0.5 0.5 1.0]  GraphicAmbientColor=[0.15 0.15 0.15 1.0]  GraphicEmissiveColor=[0.0 0.0 0.0 1.0]  GraphicShininess=75  DoExposeReferenceFrame=on  SerializedFrames=<Frames/>
  F : PMIOPort  Side=Left
  connections:
  Solid/RConn1 -- ReferenceFrame/RConn1 -- F/RConn1

== system Hexapod_dev/Spherical Joints/MotorRotor_a_3_RIGID/x91259A628_Alloy_Steel_Shoulder_Screw_1_RIGID ==
  ReferenceFrame : sm_lib/Frames and Transforms/Reference Frame
  Solid : sm_lib/Body Elements/File Solid  ExtGeomFileName=91259A628_Alloy Steel Shoulder Screw_91259A628_sldprt.STEP  UnitType=FromFile  ExtGeomFileUnits=m  StepReaderType=HEX  ExportConvexHullGeometry=off  InertiaType=Custom  BasedOnType=DensityFromFile  Density=1000  DensityUnits=kg/m^3  Mass=smiData.Solid(15).mass  MassUnits=kg  CenterOfMass=smiData.Solid(15).CoM  CenterOfMassUnits=in  MomentsOfInertia=smiData.Solid(15).MoI  MomentsOfInertiaUnits=kg*in^2  ProductsOfInertia=smiData.Solid(15).PoI  ProductsOfInertiaUnits=kg*in^2  GraphicType=FromGeometry  MarkerShape=Sphere  MarkerSize=10  GraphicVisPropType=SimpleVisualProperties  GraphicDiffuseColor=smiData.Solid(15).color  GraphicOpacity=smiData.Solid(15).opacity  GraphicSpecularColor=[0.5 0.5 0.5 1.0]  GraphicAmbientColor=[0.15 0.15 0.15 1.0]  GraphicEmissiveColor=[0.0 0.0 0.0 1.0]  GraphicShininess=75  DoExposeReferenceFrame=on  SerializedFrames=<Frames/>
  F : PMIOPort  Side=Left
  connections:
  Solid/RConn1 -- ReferenceFrame/RConn1 -- F/RConn1

== system Hexapod_dev/Spherical Joints/MotorRotor_a_3_RIGID/x91273A784_Same_Size_Thread_18_8_Stainless_Steel_Shoulder_Screw_1_RIGID ==
  ReferenceFrame : sm_lib/Frames and Transforms/Reference Frame
  Solid : sm_lib/Body Elements/File Solid  ExtGeomFileName=91273A784_Same-Size Thread 18-8 Stainless Steel Shoulder Screw_91273A784_sldprt.STEP  UnitType=FromFile  ExtGeomFileUnits=m  StepReaderType=HEX  ExportConvexHullGeometry=off  InertiaType=Custom  BasedOnType=DensityFromFile  Density=1000  DensityUnits=kg/m^3  Mass=smiData.Solid(10).mass  MassUnits=kg  CenterOfMass=smiData.Solid(10).CoM  CenterOfMassUnits=mm  MomentsOfInertia=smiData.Solid(10).MoI  MomentsOfInertiaUnits=kg*mm^2  ProductsOfInertia=smiData.Solid(10).PoI  ProductsOfInertiaUnits=kg*mm^2  GraphicType=FromGeometry  MarkerShape=Sphere  MarkerSize=10  GraphicVisPropType=SimpleVisualProperties  GraphicDiffuseColor=smiData.Solid(10).color  GraphicOpacity=smiData.Solid(10).opacity  GraphicSpecularColor=[0.5 0.5 0.5 1.0]  GraphicAmbientColor=[0.15 0.15 0.15 1.0]  GraphicEmissiveColor=[0.0 0.0 0.0 1.0]  GraphicShininess=75  DoExposeReferenceFrame=on  SerializedFrames=<Frames/>
  F : PMIOPort  Side=Left
  connections:
  Solid/RConn1 -- ReferenceFrame/RConn1 -- F/RConn1

== system Hexapod_dev/Spherical Joints/MotorRotor_a_3_RIGID/x91273A784_Same_Size_Thread_18_8_Stainless_Steel_Shoulder_Screw_2_RIGID ==
  ReferenceFrame : sm_lib/Frames and Transforms/Reference Frame
  Solid : sm_lib/Body Elements/File Solid  ExtGeomFileName=91273A784_Same-Size Thread 18-8 Stainless Steel Shoulder Screw_91273A784_sldprt.STEP  UnitType=FromFile  ExtGeomFileUnits=m  StepReaderType=HEX  ExportConvexHullGeometry=off  InertiaType=Custom  BasedOnType=DensityFromFile  Density=1000  DensityUnits=kg/m^3  Mass=smiData.Solid(10).mass  MassUnits=kg  CenterOfMass=smiData.Solid(10).CoM  CenterOfMassUnits=mm  MomentsOfInertia=smiData.Solid(10).MoI  MomentsOfInertiaUnits=kg*mm^2  ProductsOfInertia=smiData.Solid(10).PoI  ProductsOfInertiaUnits=kg*mm^2  GraphicType=FromGeometry  MarkerShape=Sphere  MarkerSize=10  GraphicVisPropType=SimpleVisualProperties  GraphicDiffuseColor=smiData.Solid(10).color  GraphicOpacity=smiData.Solid(10).opacity  GraphicSpecularColor=[0.5 0.5 0.5 1.0]  GraphicAmbientColor=[0.15 0.15 0.15 1.0]  GraphicEmissiveColor=[0.0 0.0 0.0 1.0]  GraphicShininess=75  DoExposeReferenceFrame=on  SerializedFrames=<Frames/>
  F : PMIOPort  Side=Left
  connections:
  Solid/RConn1 -- ReferenceFrame/RConn1 -- F/RConn1
